simulink model "p63_resnet50_webcam"  (R2026a)
settings: Solver=FixedStepAuto  StopTime=inf  EnableMultiTasking=on
libraries: raspberrypiAVlib x2, visionsources x1, visiongeotforms x1, deeplib x1, visiontextngfix x1
settings Model: Creator=The MathWorks, Inc.  LastModifiedBy=User
settings SolverCC: PositivePriorityOrder=on
settings OptimizationCC: PassReuseOutputArgsThreshold=0.0  MaxStackSize=200000
settings DebuggingCC: IntegerSaturationMsg=none
settings HardwareCC: ProdBitPerLong=64.0  ProdLargestAtomicInteger=LongLong  ProdLargestAtomicFloat=Double  ProdHWDeviceType=ARM Compatible->ARM Cortex-A (64-bit)
settings SFSimCC: SimTargetLang=C++
settings RTWCC: SystemTargetFile=ert.tlc  HardwareBoard=Raspberry Pi (64bit)  Toolchain=GNU GCC RPIUtils  BuildConfiguration=Faster Runs  TargetLang=C++  DLArmComputeArch=armv7  LargeConstantGeneration=WriteOnlyDNNConstantsToDataFiles  LargeConstantThreshold=64.0  Description=Embedded Coder
settings ERTTargetCC: ExtModeTransport=2.0  RootIOFormat=Structure reference  DynamicArrayContainerType=coder::array  ERTCustomFileBanners=off  SupportContinuousTime=on  SupportNonInlinedSFcns=on  SupportVariableSizeSignals=on  ModelStepFunctionPrototypeControlCompliant=off  UnsupportedSFcnMsg=none

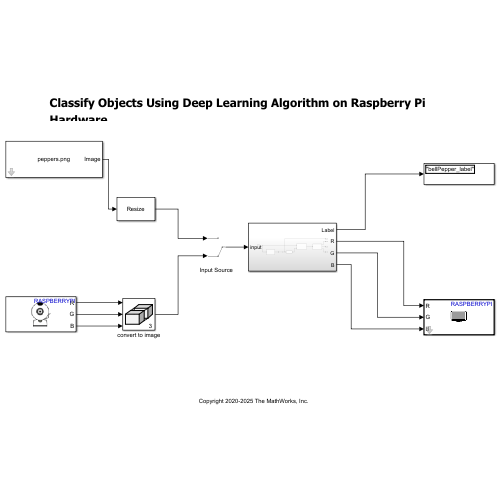
[thumbnail: Simulink's stored preview of the top-level diagram]
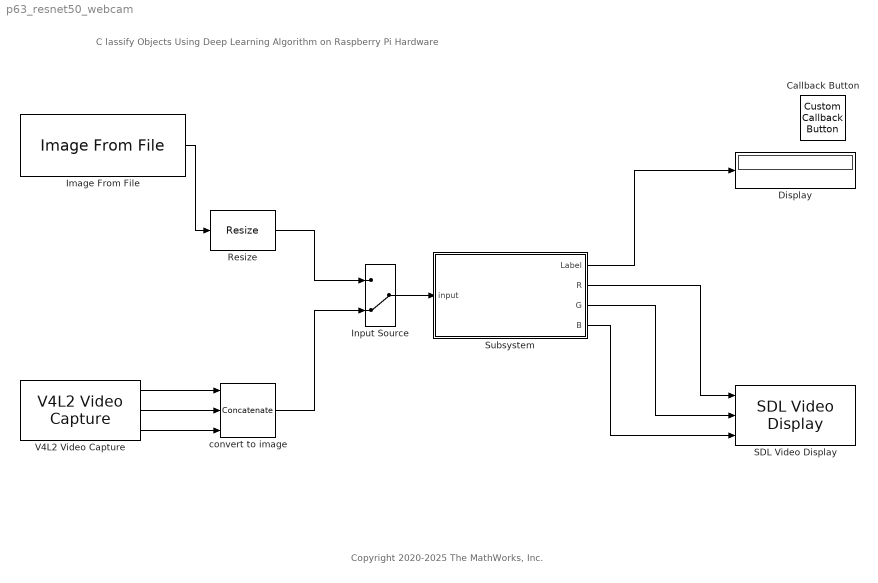
== system p63_resnet50_webcam ==
  note: C lassify Objects Using Deep Learning Algorithm on Raspberry Pi Hardware
  note: Copyright 2020-2025 The MathWorks, Inc.
  Callback Button : CustomCallbackButton  Configuration="{\"components\":[{\"name\":\"BackgroundImageComponent\",\"settings\":{\"image\":{\"size\":[0,0],\"src\":\"default\",\"srcOrientation\":\"Right\"},\"position\":[0,0,1,1]}},{\"name\":\"ButtonStateComponent\",\"settings\":{\"buttonType\":\"momentary\",\"clickFcn\":\"showExample('raspberrypi\\/ClassifyObjectsDeepLearningRaspberryPiHardwareExample')\",\"onValue\":1,\"position\":[0,0,1,1],\"pressDelay\":\"500\",\"pressFcn\":\"\",\"repeatInterval\":\"0\",\"states\":[{\"horizontalAlignment\":\"center\",\"image\":{\"position\":[0,0,1,1],\"src\":\"default\",\"srcOrientation\":\"Right\"},\"label\":{\"color\":[0.01176470588,0.01176470588,0.01176470588,1],\"icon\":{\"size\":[0,0],\"src\":\"default\",\"srcOrientation\":\"Right\"},\"iconPlacement\":\"left\",\"text\":{\"content\":\"?\"}},\"labelOffset\":[0,0],\"verticalAlignment\":\"middle\"},{\"horizontalAlignment\":\"center\",\"image\":{\"position\":[0,0,1,1],\"src\":\"default\",\"srcOrientation\":\"Right\"},\"label\":{\"color\":[0.01176470588,0.01176470588,0.01176470588,1],\"icon\":{\"size\":[0,0],\"src\":\"default\",\"srcOrientation\":\"Right\"},\"iconPlacement\":\"left\",\"text\":{\"content\":\"?\"}},\"labelOffset\":[0,0],\"verticalAlignment\":\"middle\"},{\"horizontalAlignment\":\"center\",\"image\":{\"position\":[0,0,1,1],\"src\":\"default\",\"srcOrientation\":\"Right\"},\"label\":{\"color\":[0.01176470588,0.01176470588,0.01176470588,1],\"icon\":{\"size\":[0,0],\"src\":\"default\",\"srcOrientation\":\"Right\"},\"iconPlacement\":\"left\",\"text\":{\"content\":\"?\"}},\"labelOffset\":[0,0],\"verticalAlignment\":\"middle\"},{\"horizontalAlignment\":\"center\",\"image\":{\"position\":[0,0,1,1],\"src\":\"default\",\"srcOrientation\":\"Right\"},\"label\":{\"color\":[0.01176470588,0.01176470588,0.01176470588,1],\"icon\":{\"size\":[0,0],\"src\":\"default\",\"srcOrientation\":\"Right\"},\"iconPlacement\":\"left\",\"text\":{\"content\":\"?\"}},\"labelOffset\":[0,0],\"verticalAlignment\":\"middle\"}]}},{\"name\":\"ForegroundImageComponent\",\"settings\":{\"image\":{\"size\":[0,0],\"src\":\"default\",\"srcOrientation\":\"Right\"},\"isForeground\":1,\"position\":[0,0,1,1]}}],\"derived\":{\"blockParameters\":{\"AutoActivate\":true,\"ButtonText\":\"?\",\"ButtonType\":\"Momentary\",\"ClickFcn\":\"showExample('raspberrypi\\/ClassifyObjectsDeepLearningRaspberryPiHardwareExample')\",\"OnValue\":1,\"PressDelay\":\"500\",\"PressFcn\":\"\",\"RepeatInterval\":\"0\",\"fixedAspectRatio\":\"off\"}},\"settings\":{\"BindingType\":\"standalone\",\"autoActivate\":true,\"backgroundColor\":[244,244,244,1],\"backgroundOffset\":0,\"backgroundOpacity\":1,\"fixedAspectRatio\":\"off\",\"foregroundColor\":[0.01176470588,0.01176470588,0.01176470588,1],\"migratedFromLegacy\":true,\"useBackgroundColor\":true,\"variant\":\"callback\",\"version\":\"R2025a\"},\"type\":\"Button\"}"  CustomBackgroundColor="{\"color\":[0.9568627451,0.9568627451,0.9568627451],\"show\":true}"
  Display : Display
  Image From File : visionsources/Image From File  Tag=vipblks_nd  FileName=peppers.png  Ts=inf  imagePorts=One multidimensional signal  OutPortLabels=R|G|B  ImageDataType=Inherit from input image  sdImageDataType=uint(8)  Signed=on  WordLength=16  FractionLengthMode=User-defined  FractionLength=15
  Input Source : ManualSwitch  CurrentSetting=0
  Resize : visiongeotforms/Resize  specify=Number of output rows and columns  rfactor=[200 150]  outCols=25  outRows=25  outRowsCols=[320 240]  interp_method=Bilinear  antialias=on  useROI=off  roiFlag=off  roundingMode=Nearest  overflowMode=on  prodOutputMode=Binary point scaling  prodOutputWordLength=32  prodOutputFracLength=10
      settings: LockScale=on
  SDL Video Display : raspberrypiAVlib/SDL Video Display  title=SDL Video Display  pixelFormat=RGB  pixelOrder=Planar  rowMajor=on  blockPlatform=Raspberry Pi
  Subsystem : Subsystem
  V4L2 Video Capture : raspberrypiAVlib/V4L2 Video Capture  DeviceName=/dev/video0  Resolution=320x240  CustomResolution=[ 320, 240 ]  PixelFormat=RGB  SampleTime=0.1  pixelOrder=planar  simOutput=Colorbars  imSizeSelection=320x240  imSize=[640, 480]  roi=[0, 0, 640, 480]  m_devName='/dev/video0'  blockPlatform=LINUX  HorizontalFlip=off  VerticalFlip=off  Brightness=0.5  Saturation=0.5  Contrast=0.5  Sharpness=0.5  CameraPan=0  CameraTilt=0  CameraZoom=0.5  EnableManualFocus=on  ManualFocus=0.5
  convert to image : Concatenate  NumInputs=3  Mode=Multidimensional array  ConcatenateDimension=3
  wires:
  Subsystem/3(G) -> SDL Video Display/2
  Subsystem/4(B) -> SDL Video Display/3
  V4L2 Video Capture/1 -> convert to image/1
  V4L2 Video Capture/2 -> convert to image/2
  Input Source/1 -> Subsystem/1(input)
  convert to image/1 -> Input Source/2
  V4L2 Video Capture/3 -> convert to image/3
  Resize/1 -> Input Source/1
  Subsystem/1(Label) -> Display/1
  Image From File/1 -> Resize/1
  Subsystem/2(R) -> SDL Video Display/1

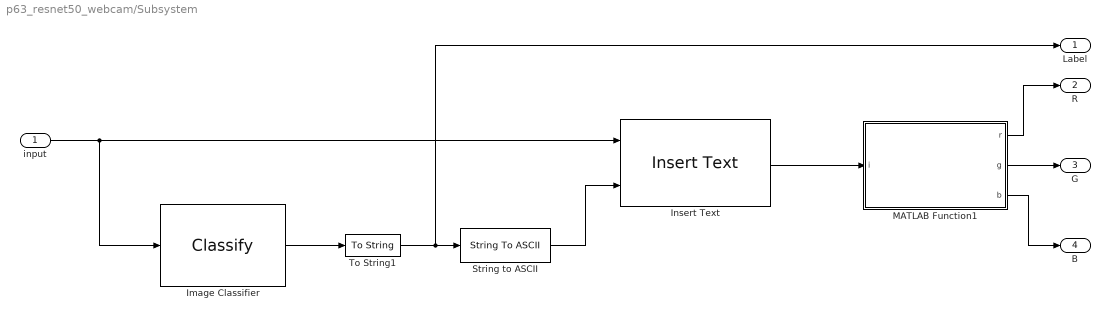
== system p63_resnet50_webcam/Subsystem ==
  input : Inport
  Image Classifier : deeplib/Classify  Network=Network from MATLAB function  NetworkFunction=resnet50  NetworkFilePath=untitled.mat  NetworkClassesVariable=classNames  MiniBatchSize=128  SimulateUsing=Auto mode  ResizeInput=on  InputDataFormats={' ',' '}  Classification=on  Predictions=off  ForceInterpretedSim=off  PredictMode=All probabilities and labels  K=5  LastKnownNetworkFilePath=''  LastKnownNetworkTimeStamp=0
  Insert Text : visiontextngfix/Insert Text  inputType=Obsolete  theText='%s'  getTextLocFrom=Specify via dialog  textLoc=[1 1]  getTextColorFrom=Specify via dialog  textColor=[255,255,0]  getTextIntensityFrom=Specify via dialog  textIntensity=0  getTextOpacityFrom=Specify via dialog  textOpacity=1.0  dummyVar2=0  dummyVar3=0  dummyVar4=0  imagePorts=One multidimensional signal  isInputTransposed=on  fontFace=LucidaSansRegular  dummyVar1=0  blockFontSize=18  antiAliased=off
  MATLAB Function1 : MATLAB Function  TreatAsAtomicUnit=on
  String to ASCII : StringToASCII
  To String1 : ToString
  Label : Outport
  R : Outport  Port=2
  G : Outport  Port=3
  B : Outport  Port=4
  wires:
  input/1 -> Image Classifier/1, Insert Text/1
  MATLAB Function1/2(g) -> G/1
  MATLAB Function1/1(r) -> R/1
  MATLAB Function1/3(b) -> B/1
  Image Classifier/1 -> To String1/1
  Insert Text/1 -> MATLAB Function1/1(i)
  To String1/1 -> Label/1, String to ASCII/1
  String to ASCII/1 -> Insert Text/2

== matlab function p63_resnet50_webcam/Subsystem/MATLAB Function1 ==
  data: i input; r output; g output; b output
function [r,g,b] = ImageToRGB(i)
%#codegen
r =i(:,:,1);
g =i(:,:,2);
b =i(:,:,3);
end
